simulink model "Cable_with_M_Inductance_Modelling_Study"  (R2024b)
settings: Solver=FixedStepDiscrete  StartTime=0.0  StopTime=5  FixedStep=1e-6  RelTol=1e-3
values from neighbouring files (symbols this model uses):
  Ccs1 = 733.62e-12    (= 7.3362e-10)    [Cable_Data_Inductance_Study.m]
  Ccs2 = 733.62e-12    (= 7.3362e-10)    [Cable_Data_Inductance_Study.m]
  Csg1 = 216.23e-12    (= 2.1623e-10)    [Cable_Data_Inductance_Study.m]
  Csg2 = 216.23e-12    (= 2.1623e-10)    [Cable_Data_Inductance_Study.m]
  Css = 93.23e-12    (= 9.323e-11)    [Cable_Data_Inductance_Study.m]
  L35 = 0.098e-6    (= 9.8e-08)    [Cable_Data_Inductance_Study.m]
  Lc1_total = Lc1 + Mcs1    (= 2.72e-07)    [Cable_Data_Inductance_Study.m]
  Lc2_total = Lc2 + Mcs2    (= 2.72e-07)    [Cable_Data_Inductance_Study.m]
  Len35_batt1_HVJB1_neg = 0.600    (= 0.6)    [Cable_Data_Inductance_Study.m]
  Len35_batt1_HVJB1_pos = 0.750    (= 0.75)    [Cable_Data_Inductance_Study.m]
  Len_parallel = min(Len35_batt1_HVJB1_pos,Len35_batt1_HVJB1_neg)    [Cable_Data_Inductance_Study.m]
  Ls1_eff = Ls1 + Mss_cal    [Cable_Data_Inductance_Study.m]
  Ls2_eff = Ls2 + Mss_cal    [Cable_Data_Inductance_Study.m]
  Mcs1 = 0.180e-6    (= 1.8e-07)    [Cable_Data_Inductance_Study.m]
  Mcs2 = 0.180e-6    (= 1.8e-07)    [Cable_Data_Inductance_Study.m]
  Rc1 = 0.38e-3    (= 0.00038)    [Cable_Data_Inductance_Study.m]
  Rc2 = 0.38e-3    (= 0.00038)    [Cable_Data_Inductance_Study.m]
  Rs1 = 2.55e-3    (= 0.00255)    [Cable_Data_Inductance_Study.m]
  Rs2 = 2.55e-3    (= 0.00255)    [Cable_Data_Inductance_Study.m]
undefined symbols (not defined in the file or in its folder): DiscIntNeverNeededParam, Lns95, Lps95
libraries: spsSeriesRLCBranchLib x18, spsCurrentMeasurementLib x7, spsMultimeterLib x6, spsVoltageMeasurementLib x5, eeGeneralControl x2, spsMutualInductanceLib x2, spsVariableResistorLib x1, spsGroundLib x1, spsDCVoltageSourceLib x1, spspowerguiLib x1
settings Model: PauseTimes=9  SnapshotBufferSize=100000000  SnapshotInterval=100  Creator=SUDHAK1  LastModifiedBy=SUDHAK1

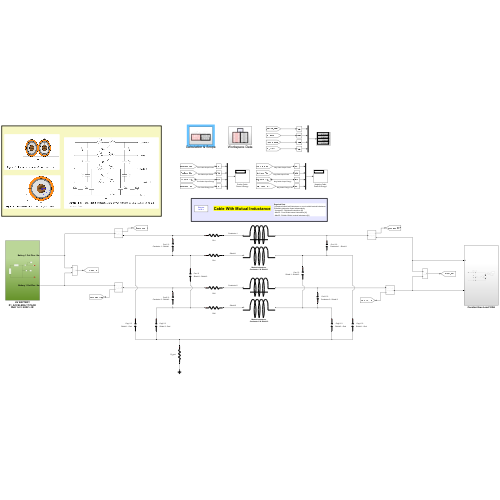
[thumbnail: Simulink's stored preview of the top-level diagram]
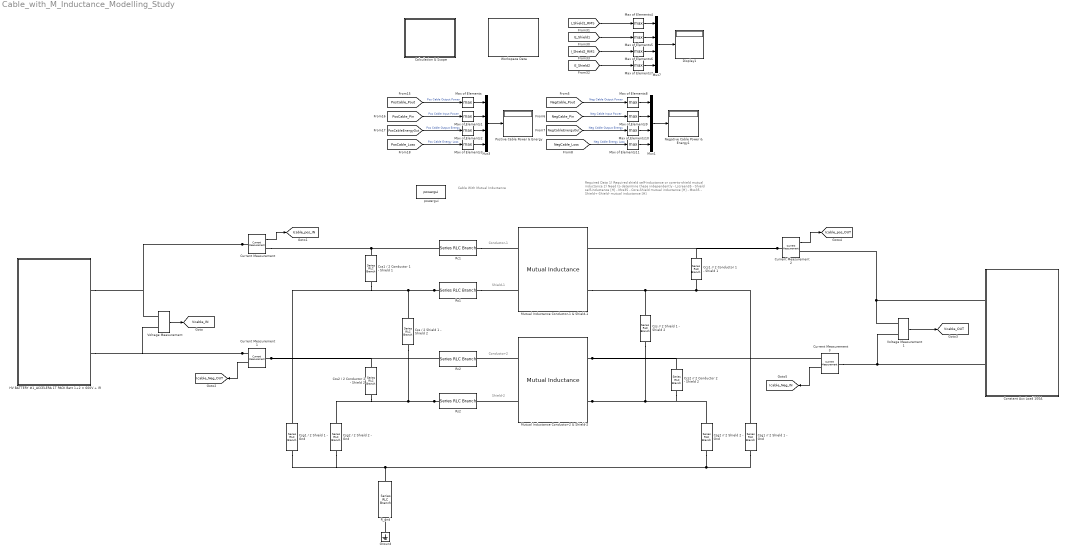
== system Cable_with_M_Inductance_Modelling_Study ==
  note: Cable With Mutual Inductance
  note: Shield-2
  note: Conductor-1
  note: Shield-1
  note: Required Data
      | 1) Required shield self-inductance or core-to-shield mutual inductance
      | 2) Need to determine these independently
      | - Lscreen35 - Shield self-inductance [H]
      | - Mcs35 - Core-Shield mutual inductance [H]
      | - Mss35 - Shield+-Shield- mutual inductance [H]
  note: Conductor-2
  " Ccs1 // 2 Conductor 1 - Shield 1" : spsSeriesRLCBranchLib/Series RLC Branch  LConnTagsString=__new0  RConnTagsString=__new0  BranchType=C  Resistance=1  Inductance=1e-3  SetiL0=off  InitialCurrent=0  Capacitance=(Ccs1/2)*Len35_batt1_HVJB1_pos  Setx0=off  InitialVoltage=0  Measurements=None
  " Ccs2 // 2 Conductor 2 - Shield 2" : spsSeriesRLCBranchLib/Series RLC Branch  LConnTagsString=__new0  RConnTagsString=__new0  BranchType=C  Resistance=1  Inductance=1e-3  SetiL0=off  InitialCurrent=0  Capacitance=(Ccs2/2)*Len35_batt1_HVJB1_neg  Setx0=off  InitialVoltage=0  Measurements=None
  " Csg1 // 2 Shield 1 - Gnd" : spsSeriesRLCBranchLib/Series RLC Branch  LConnTagsString=__new0  RConnTagsString=__new0  BranchType=C  Resistance=1  Inductance=1e-3  SetiL0=off  InitialCurrent=0  Capacitance=(Csg1/2)*Len35_batt1_HVJB1_pos  Setx0=off  InitialVoltage=0  Measurements=Branch voltage and current
  " Csg2 // 2 Shield 2 - Gnd" : spsSeriesRLCBranchLib/Series RLC Branch  LConnTagsString=__new0  RConnTagsString=__new0  BranchType=C  Resistance=1  Inductance=1e-3  SetiL0=off  InitialCurrent=0  Capacitance=(Csg2/2)*Len35_batt1_HVJB1_neg  Setx0=off  InitialVoltage=0  Measurements=Branch voltage and current
  " Css // 2 Shield 1 - Shield 2" : spsSeriesRLCBranchLib/Series RLC Branch  LConnTagsString=__new0  RConnTagsString=__new0  BranchType=C  Resistance=1  Inductance=1e-3  SetiL0=off  InitialCurrent=0  Capacitance=(Css/2)*Len_parallel  Setx0=off  InitialVoltage=0  Measurements=Branch voltage and current
  Calculation & Scope : Subsystem
  Ccs1 / 2 Conductor 1 - Shield 1 : spsSeriesRLCBranchLib/Series RLC Branch  LConnTagsString=__new0  RConnTagsString=__new0  BranchType=C  Resistance=1  Inductance=1e-3  SetiL0=off  InitialCurrent=0  Capacitance=(Ccs1/2)*Len35_batt1_HVJB1_pos  Setx0=off  InitialVoltage=0  Measurements=None
  Ccs2 / 2 Conductor 2 - Shield 2 : spsSeriesRLCBranchLib/Series RLC Branch  LConnTagsString=__new0  RConnTagsString=__new0  BranchType=C  Resistance=1  Inductance=1e-3  SetiL0=off  InitialCurrent=0  Capacitance=(Ccs2/2)*Len35_batt1_HVJB1_neg  Setx0=off  InitialVoltage=0  Measurements=None
  Constant Aux Load 100A : Subsystem
  Csg1 / 2 Shield 1 - Gnd : spsSeriesRLCBranchLib/Series RLC Branch  LConnTagsString=__new0  RConnTagsString=__new0  BranchType=C  Resistance=1  Inductance=1e-3  SetiL0=off  InitialCurrent=0  Capacitance=(Csg1/2)*Len35_batt1_HVJB1_pos  Setx0=off  InitialVoltage=0  Measurements=Branch voltage and current
  Csg2 / 2 Shield 2 - Gnd : spsSeriesRLCBranchLib/Series RLC Branch  LConnTagsString=__new0  RConnTagsString=__new0  BranchType=C  Resistance=1  Inductance=1e-3  SetiL0=off  InitialCurrent=0  Capacitance=(Csg2/2)*Len35_batt1_HVJB1_neg  Setx0=off  InitialVoltage=0  Measurements=Branch voltage and current
  Css / 2 Shield 1 - Shield 2 : spsSeriesRLCBranchLib/Series RLC Branch  LConnTagsString=__new0  RConnTagsString=__new0  BranchType=C  Resistance=1  Inductance=1e-3  SetiL0=off  InitialCurrent=0  Capacitance=(Css/2)*Len_parallel  Setx0=off  InitialVoltage=0  Measurements=Branch voltage and current
  Current Measurement{,1..3} (4 alike) : spsCurrentMeasurementLib/Current Measurement  PhasorSimulation=off  OutputType=Complex  PSBequivalent=0
  Display1 : Display
  Ground : spsGroundLib/Ground  LConnTagsString=a
  HV BATTERY #1_ACCELERA 1T PACK Batt 1+2 = 600V + IR : Subsystem
  Max of Elements{,1..11} (12 alike) : MinMax  Function=max
  Mutual Inductance Conductor-1 & Shield-1 : spsMutualInductanceLib/Mutual Inductance  LConnTagsString=a|b  RConnTagsString=A|B  TypeOfMutual=Two or three windings with equal mutual terms  NumberOfWindings=3  SelfImpedance1=[0 Lc1_total*Len35_batt1_HVJB1_pos]  SelfImpedance2=[0 Ls1_eff*Len35_batt1_HVJB1_pos]  ThreeWindings=off  SelfImpedance3=[ 1.1 1.1e-03]  MutualImpedance=[0 Mcs1*Len35_batt1_HVJB1_pos]  InductanceMatrix="[1.0 0.9  0.9 ;  0.9 1.0  0.9;  0.9 0.9 1.0 ] * 1e-3"  ResistanceMatrix="[1.0 0.9  0.9 ;  0.9 1.0  0.9;  0.9 0.9 1.0 ]"  Measurements=Winding voltages and currents
      settings: LibrarySourceBlock=sps_lib/Passives/Mutual Inductance
  Mutual Inductance Conductor-2 & Shield-2 : spsMutualInductanceLib/Mutual Inductance  LConnTagsString=a|b  RConnTagsString=A|B  TypeOfMutual=Two or three windings with equal mutual terms  NumberOfWindings=3  SelfImpedance1=[0 Lc2_total*Len35_batt1_HVJB1_neg]  SelfImpedance2=[0 Ls2_eff*Len35_batt1_HVJB1_neg]  ThreeWindings=off  SelfImpedance3=[ 1.1 1.1e-03]  MutualImpedance=[0 Mcs2*Len35_batt1_HVJB1_neg]  InductanceMatrix="[1.0 0.9  0.9 ;  0.9 1.0  0.9;  0.9 0.9 1.0 ] * 1e-3"  ResistanceMatrix="[1.0 0.9  0.9 ;  0.9 1.0  0.9;  0.9 0.9 1.0 ]"  Measurements=Winding voltages and currents
      settings: LibrarySourceBlock=sps_lib/Passives/Mutual Inductance
  Mux1 : Mux
  Mux3 : Mux
  Mux7 : Mux
  Negative Cable Power & Energy1 : Display
  Postive Cable Power & Energy : Display
  R_gnd : spsSeriesRLCBranchLib/Series RLC Branch  LConnTagsString=__new0  RConnTagsString=__new0  BranchType=R  Resistance=10e-03  Inductance=1e-3  SetiL0=off  InitialCurrent=0  Capacitance=1e-6  Setx0=off  InitialVoltage=0  Measurements=Branch voltage and current
  Rc1 : spsSeriesRLCBranchLib/Series RLC Branch  LConnTagsString=__new0  RConnTagsString=__new0  BranchType=R  Resistance=Rc1*Len35_batt1_HVJB1_pos  Inductance=L35*Len35_batt1_HVJB1_pos  SetiL0=off  InitialCurrent=0  Capacitance=1e-6  Setx0=off  InitialVoltage=0  Measurements=None
  Rc2 : spsSeriesRLCBranchLib/Series RLC Branch  LConnTagsString=__new0  RConnTagsString=__new0  BranchType=R  Resistance=Rc2*Len35_batt1_HVJB1_neg  Inductance=L35*Len35_batt1_HVJB1_pos  SetiL0=off  InitialCurrent=0  Capacitance=1e-6  Setx0=off  InitialVoltage=0  Measurements=None
  Rs1 : spsSeriesRLCBranchLib/Series RLC Branch  LConnTagsString=__new0  RConnTagsString=__new0  BranchType=R  Resistance=Rs1*Len35_batt1_HVJB1_pos  Inductance=Lps95*3.270  SetiL0=off  InitialCurrent=0  Capacitance=1e-6  Setx0=off  InitialVoltage=0  Measurements=None
  Rs2 : spsSeriesRLCBranchLib/Series RLC Branch  LConnTagsString=__new0  RConnTagsString=__new0  BranchType=R  Resistance=Rs2*Len35_batt1_HVJB1_neg  Inductance=Lns95*3.305  SetiL0=off  InitialCurrent=0  Capacitance=1e-6  Setx0=off  InitialVoltage=0  Measurements=None
  Voltage Measurement : spsVoltageMeasurementLib/Voltage Measurement  PhasorSimulation=off  OutputType=Complex  PSBequivalent=0
  Voltage Measurement1 : spsVoltageMeasurementLib/Voltage Measurement  PhasorSimulation=off  OutputType=Complex  PSBequivalent=0
  Workspace Data : Subsystem
  powergui : spspowerguiLib/powergui  Priority=1  SimulationMode=Discrete  SampleTime=1e-6  frequency=60  Iterations=50  frequencyindice=0  Pbase=100e6  ErrMax=1e-4  UnitsV=kV  UnitsW=MW  buscounter=0  FunctionMessages=off  echomessages=off  EnableUseOfTLC=off  CurrentSourceSwitches=off  DisableSnubberDevices=off  DisableRonSwitches=off  DisableVfSwitches=off  DisplayEquations=off  AutomaticDiscreteSolvers=off  SolverType=Tustin/Backward Euler (TBE)  Interpol=off  ExternalGateDelay=off  methode=off  Ts=100  x0status=blocks  SPID=on  SwTol=0  HookPort=off  NonlinearTolerance=1e-4  nMaxIteration=100  ContinueOnMaxIteration=off  RestoreLinks=warning  ResistiveCurrentMeasurement=off  Frange=[0:2:500]  Ylog=off  Xlog=on  ShowGrid=off  save=off  variable=ZData  structure=0  ZoomFFT=off  StartTime=0.0  cycles=1  DisplayStyle=1  fundamental=60  FreqAxis=off  MaxFrequency=1000  frequencyindicesteady=1  RmsSteady=1  display=off
  tag scope: Icable_Neg_IN=global, Icable_Neg_OUT=global, Icable_pos_IN=global, Icable_pos_OUT=global, Vcable_IN=global, Vcable_OUT=global
  wires:
  Current Measurement2/1 -> [Icable_pos_OUT]
  Current Measurement3/1 -> [Icable_Neg_IN]
  Voltage Measurement1/1 -> [Vcable_OUT]
  Current Measurement1/1 -> [Icable_Neg_OUT]
  Voltage Measurement/1 -> [Vcable_IN]
  Current Measurement/1 -> [Icable_pos_IN]
  Max of Elements4/1 -> Mux7/1
  Max of Elements5/1 -> Mux7/2
  Mux7/1 -> Display1/1
  [I_Shield1_RMS] -> Max of Elements4/1
  [E_Shield1] -> Max of Elements5/1
  Max of Elements6/1 -> Mux7/3
  Max of Elements7/1 -> Mux7/4
  [I_Shield2_RMS] -> Max of Elements6/1
  [E_Shield2] -> Max of Elements7/1
  [NegCable_Loss] -> Max of Elements11/1  "Neg Cable Energy Loss"
  [NegCableEnergyOut] -> Max of Elements10/1  "Neg Cable Output Energy"
  [PosCable_Loss] -> Max of Elements3/1  "Pos Cable Energy Loss"
  [PosCableEnergyOut] -> Max of Elements2/1  "Pos Cable Output Energy"
  [PosCable_Pout] -> Max of Elements/1  "Pos Cable Output Power"
  [NegCable_Pout] -> Max of Elements8/1  "Neg Cable Output Power"
  [NegCable_Pin] -> Max of Elements9/1  "Neg Cable Input Power"
  [PosCable_Pin] -> Max of Elements1/1  "Pos Cable Input Power"
  Max of Elements3/1 -> Mux3/4
  Max of Elements/1 -> Mux3/1
  Mux3/1 -> Postive Cable Power & Energy/1
  Max of Elements1/1 -> Mux3/2
  Max of Elements2/1 -> Mux3/3
  Max of Elements10/1 -> Mux1/3
  Max of Elements9/1 -> Mux1/2
  Max of Elements8/1 -> Mux1/1
  Mux1/1 -> Negative Cable Power & Energy1/1
  Max of Elements11/1 -> Mux1/4
  connections:
  Mutual Inductance Conductor-2 & Shield-2/RConn1 -- Current Measurement3/RConn1 -- " Ccs2 // 2 Conductor 2 - Shield 2"/RConn1
  Current Measurement1/RConn1 -- HV BATTERY #1_ACCELERA 1T PACK Batt 1+2 = 600V + IR/RConn2 -- Voltage Measurement/LConn2
  Current Measurement1/LConn1 -- Rc2/LConn1 -- Ccs2 / 2 Conductor 2 - Shield 2/LConn1
  Voltage Measurement1/LConn1 -- Constant Aux Load 100A/RConn1 -- Current Measurement2/RConn1
  Rs1/LConn1 -- Ccs1 / 2 Conductor 1 - Shield 1/RConn1 -- Csg1 / 2 Shield 1 - Gnd/LConn1 -- Css / 2 Shield 1 - Shield 2/LConn1
  Current Measurement/LConn1 -- Voltage Measurement/LConn1 -- HV BATTERY #1_ACCELERA 1T PACK Batt 1+2 = 600V + IR/RConn1
  Rs2/LConn1 -- Csg2 / 2 Shield 2 - Gnd/LConn1 -- Ccs2 / 2 Conductor 2 - Shield 2/RConn1 -- Css / 2 Shield 1 - Shield 2/RConn1
  Mutual Inductance Conductor-2 & Shield-2/RConn2 -- " Csg2 // 2 Shield 2 - Gnd"/LConn1 -- " Ccs2 // 2 Conductor 2 - Shield 2"/LConn1 -- " Css // 2 Shield 1 - Shield 2"/RConn1
  R_gnd/LConn1 -- Csg2 / 2 Shield 2 - Gnd/RConn1 -- Csg1 / 2 Shield 1 - Gnd/RConn1 -- " Csg2 // 2 Shield 2 - Gnd"/RConn1 -- " Csg1 // 2 Shield 1 - Gnd"/RConn1
  Current Measurement/RConn1 -- Rc1/LConn1 -- Ccs1 / 2 Conductor 1 - Shield 1/LConn1
  " Css // 2 Shield 1 - Shield 2"/LConn1 -- Mutual Inductance Conductor-1 & Shield-1/RConn2 -- " Csg1 // 2 Shield 1 - Gnd"/LConn1 -- " Ccs1 // 2 Conductor 1 - Shield 1"/RConn1
  Current Measurement3/LConn1 -- Constant Aux Load 100A/RConn2 -- Voltage Measurement1/LConn2
  Current Measurement2/LConn1 -- Mutual Inductance Conductor-1 & Shield-1/RConn1 -- " Ccs1 // 2 Conductor 1 - Shield 1"/LConn1
  Rs1/RConn1 -- Mutual Inductance Conductor-1 & Shield-1/LConn2
  Mutual Inductance Conductor-2 & Shield-2/LConn1 -- Rc2/RConn1
  Rc1/RConn1 -- Mutual Inductance Conductor-1 & Shield-1/LConn1
  Ground/LConn1 -- R_gnd/RConn1
  Mutual Inductance Conductor-2 & Shield-2/LConn2 -- Rs2/RConn1

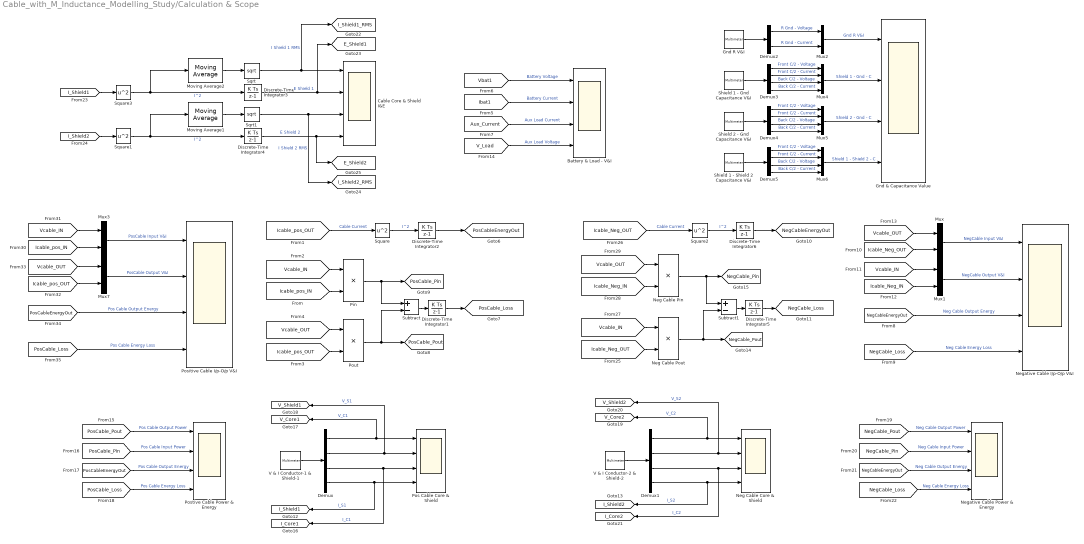
== system Cable_with_M_Inductance_Modelling_Study/Calculation & Scope ==
  Battery & Load - V&I : Scope  NumInputPorts=4
  Cable Core & Shield  I&E : Scope  NumInputPorts=4
  Demux{,1,3..5} (5 alike) : Demux
  Demux2 : Demux  Outputs=2
  Discrete-Time Integrator{1..6} (6 alike) : DiscreteIntegrator  SampleTime=-1  ICPrevOutput=DiscIntNeverNeededParam  ICPrevScaledInput=DiscIntNeverNeededParam
  Gnd & Capacitance Value : Scope  NumInputPorts=4
  Gnd R V&I : spsMultimeterLib/Multimeter  L=22  sel=[7 18]  yselected={}  Gain=[1 1]  OutputType=Complex  PlotAtSimulationStop=off  PhasorSimulation=off
  Moving Average1 : eeGeneralControl/Moving Average  VariantControl=Variant1  LabelModeActiveChoice=Discrete  f=60  x0=0  BufferSize=8192  Ts=-1
      settings: LibrarySourceBlock=ee_sl_lib/General Control/Moving Average
  Moving Average2 : eeGeneralControl/Moving Average  VariantControl=Variant1  LabelModeActiveChoice=Discrete  f=60  x0=0  BufferSize=8192  Ts=-1
      settings: LibrarySourceBlock=ee_sl_lib/General Control/Moving Average
  Mux{,1..3,7} (5 alike) : Mux  Inputs=2
  Mux4 : Mux
  Mux5 : Mux
  Mux6 : Mux
  Neg Cable Core & Shield : Scope  NumInputPorts=4
  Neg Cable Pin : Product
  Neg Cable Pout : Product
  Negative Cable Power & Energy : Scope  NumInputPorts=4
  Negative Cable I/p-O/p V&I : Scope  NumInputPorts=4
  Pin : Product
  Pos Cable Core & Shield : Scope  NumInputPorts=4
  Positive Cable I/p-O/p V&I : Scope  NumInputPorts=4
  Postive Cable Power & Energy : Scope  NumInputPorts=4
  Pout : Product
  Shield 1 - Gnd Capacitance V&I : spsMultimeterLib/Multimeter  L=22  sel=[4 15 1 12]  yselected={}  Gain=[1 1 1 1]  OutputType=Complex  PlotAtSimulationStop=off  PhasorSimulation=off
  Shield 1 - Shield 2 Capacitance V&I : spsMultimeterLib/Multimeter  L=22  sel=[6 17 3 14]  yselected={}  Gain=[1 1 1 1]  OutputType=Complex  PlotAtSimulationStop=off  PhasorSimulation=off
  Shield 2 - Gnd Capacitance V&I : spsMultimeterLib/Multimeter  L=22  sel=[5 16 2 13]  yselected={}  Gain=[1 1 1 1]  OutputType=Complex  PlotAtSimulationStop=off  PhasorSimulation=off
  Sqrt : Sqrt
  Sqrt1 : Sqrt
  Square{,1..3} (4 alike) : Math  Operator=square
  Subtract : Sum  Inputs=+-
  Subtract1 : Sum  Inputs=+-
  V & I Conductor-1 & Shield-1 : spsMultimeterLib/Multimeter  L=22  sel=[8 9 19 20]  yselected={}  Gain=[1 1 1 1]  OutputType=Complex  PlotAtSimulationStop=off  PhasorSimulation=off
  V & I Conductor-2 & Shield-2 : spsMultimeterLib/Multimeter  L=22  sel=[10 11 21 22]  yselected={}  Gain=[1 1 1 1]  OutputType=Complex  PlotAtSimulationStop=off  PhasorSimulation=off
  tag scope: E_Shield1=global, E_Shield2=global, I_Core1=global, I_Core2=global, I_Shield1=global, I_Shield1_RMS=global, I_Shield2=global, I_Shield2_RMS=global, NegCableEnergyOut=global, NegCable_Loss=global, NegCable_Pin=global, NegCable_Pout=global, PosCableEnergyOut=global, PosCable_Loss=global, PosCable_Pin=global, PosCable_Pout=global, V_Core1=global, V_Core2=global, V_Shield1=global, V_Shield2=global
  wires:
  [NegCableEnergyOut] -> Negative Cable I/p-O/p V&I/3  "Neg Cable Output Energy"
  Moving Average2/1 -> Sqrt/1
  Mux6/1 -> Gnd & Capacitance Value/4  "Shield 1 - Shield 2 - C"
  Square/1 -> Discrete-Time Integrator2/1  "I^2"
  Demux4/2 -> Mux5/2  "Front C/2 - Current"
  Mux4/1 -> Gnd & Capacitance Value/2  "Shield 1 - Gnd - C"
  [Icable_pos_IN] -> Pin/2
  Demux/4 -> [I_Shield1], Pos Cable Core & Shield/4  "I_S1"
  [PosCableEnergyOut] -> Postive Cable Power & Energy/3  "Pos Cable Output Energy"
  Demux5/2 -> Mux6/2  "Front C/2 - Current"
  Shield 1 - Shield 2 Capacitance V&I/1 -> Demux5/1
  Mux5/1 -> Gnd & Capacitance Value/3  "Shield 2 - Gnd - C"
  Shield 2 - Gnd Capacitance V&I/1 -> Demux4/1
  [Icable_pos_OUT] -> Pout/2
  Demux3/2 -> Mux4/2  "Front C/2 - Current"
  Demux1/2 -> Neg Cable Core & Shield/2, [V_Shield2]  "V_S2"
  [Icable_pos_OUT] -> Square/1  "Cable Current"
  Moving Average1/1 -> Sqrt1/1
  Discrete-Time Integrator3/1 -> [E_Shield1], Cable Core & Shield  I&E/2  "E Shield 1"
  Demux1/1 -> [V_Core2], Neg Cable Core & Shield/1  "V_C2"
  Demux/1 -> Pos Cable Core & Shield/1, [V_Core1]  "V_C1"
  Pin/1 -> [PosCable_Pin], Subtract/1
  Demux4/4 -> Mux5/4  "Back C/2 - Current"
  [Vcable_OUT] -> Pout/1
  Mux/1 -> Negative Cable I/p-O/p V&I/1  "NegCable Input V&I"
  V & I Conductor-1 & Shield-1/1 -> Demux/1
  [Aux_Current] -> Battery & Load - V&I/3  "Aux Load Current"
  [V_Load] -> Battery & Load - V&I/4  "Aux Load Voltage"
  [Icable_Neg_OUT] -> Mux/2
  Demux4/1 -> Mux5/1  "Front C/2 - Voltage"
  Discrete-Time Integrator4/1 -> Cable Core & Shield  I&E/4, [E_Shield2]  "E Shield 2"
  Square3/1 -> Discrete-Time Integrator3/1, Moving Average2/1  "I^2"
  [I_Shield1] -> Square3/1
  [Vbat1] -> Battery & Load - V&I/1  "Battery Voltage"
  Discrete-Time Integrator1/1 -> [PosCable_Loss]
  Sqrt1/1 -> Cable Core & Shield  I&E/3, [I_Shield2_RMS]  "I Shield 2 RMS"
  Demux5/4 -> Mux6/4  "Back C/2 - Current"
  Demux4/3 -> Mux5/3  "Back C/2 - Voltage"
  [Vcable_IN] -> Neg Cable Pout/1
  Demux2/2 -> Mux2/2  "R Gnd - Current"
  [NegCable_Loss] -> Negative Cable I/p-O/p V&I/4  "Neg Cable Energy Loss"
  Subtract/1 -> Discrete-Time Integrator1/1
  Demux5/1 -> Mux6/1  "Front C/2 - Voltage"
  Shield 1 - Gnd Capacitance V&I/1 -> Demux3/1
  Pout/1 -> Subtract/2, [PosCable_Pout]
  [Icable_Neg_OUT] -> Square2/1  "Cable Current"
  [PosCable_Pin] -> Postive Cable Power & Energy/2  "Pos Cable Input Power"
  Demux/2 -> Pos Cable Core & Shield/2, [V_Shield1]  "V_S1"
  Demux5/3 -> Mux6/3  "Back C/2 - Voltage"
  Demux2/1 -> Mux2/1  "R Gnd - Voltage"
  Mux2/1 -> Gnd & Capacitance Value/1  "Gnd R V&I"
  [I_Shield2] -> Square1/1
  Demux/3 -> [I_Core1], Pos Cable Core & Shield/3  "I_C1"
  Mux1/1 -> Negative Cable I/p-O/p V&I/2  "NegCable Output V&I"
  Demux3/3 -> Mux4/3  "Back C/2 - Voltage"
  Discrete-Time Integrator2/1 -> [PosCableEnergyOut]
  [Vcable_IN] -> Pin/1
  Gnd R V&I/1 -> Demux2/1
  Demux3/1 -> Mux4/1  "Front C/2 - Voltage"
  Square1/1 -> Discrete-Time Integrator4/1, Moving Average1/1  "I^2"
  [Icable_Neg_IN] -> Mux1/2
  [PosCable_Pout] -> Postive Cable Power & Energy/1  "Pos Cable Output Power"
  [PosCable_Loss] -> Postive Cable Power & Energy/4  "Pos Cable Energy Loss"
  Demux1/3 -> [I_Core2], Neg Cable Core & Shield/3  "I_C2"
  Demux1/4 -> [I_Shield2], Neg Cable Core & Shield/4  "I_S2"
  V & I Conductor-2 & Shield-2/1 -> Demux1/1
  [Ibat1] -> Battery & Load - V&I/2  "Battery Current"
  Sqrt/1 -> Cable Core & Shield  I&E/1, [I_Shield1_RMS]  "I Shield 1 RMS"
  Demux3/4 -> Mux4/4  "Back C/2 - Current"
  Subtract1/1 -> Discrete-Time Integrator5/1
  Discrete-Time Integrator5/1 -> [NegCable_Loss]
  Neg Cable Pout/1 -> Subtract1/2, [NegCable_Pout]
  Discrete-Time Integrator6/1 -> [NegCableEnergyOut]
  [Vcable_OUT] -> Neg Cable Pin/1
  Neg Cable Pin/1 -> Subtract1/1, [NegCable_Pin]
  [Icable_Neg_IN] -> Neg Cable Pin/2
  [Icable_Neg_OUT] -> Neg Cable Pout/2
  Square2/1 -> Discrete-Time Integrator6/1  "I^2"
  [NegCable_Loss] -> Negative Cable Power & Energy/4  "Neg Cable Energy Loss"
  [NegCableEnergyOut] -> Negative Cable Power & Energy/3  "Neg Cable Output Energy"
  [NegCable_Pout] -> Negative Cable Power & Energy/1  "Neg Cable Output Power"
  [NegCable_Pin] -> Negative Cable Power & Energy/2  "Neg Cable Input Power"
  [Icable_pos_IN] -> Mux3/2
  [Vcable_IN] -> Mux3/1
  [Icable_pos_OUT] -> Mux7/2
  [PosCable_Loss] -> Positive Cable I/p-O/p V&I/4  "Pos Cable Energy Loss"
  Mux3/1 -> Positive Cable I/p-O/p V&I/1  "PosCable Input V&I"
  Mux7/1 -> Positive Cable I/p-O/p V&I/2  "PosCable Output V&I"
  [Vcable_OUT] -> Mux7/1
  [PosCableEnergyOut] -> Positive Cable I/p-O/p V&I/3  "Pos Cable Output Energy"
  [Vcable_IN] -> Mux1/1
  [Vcable_OUT] -> Mux/1

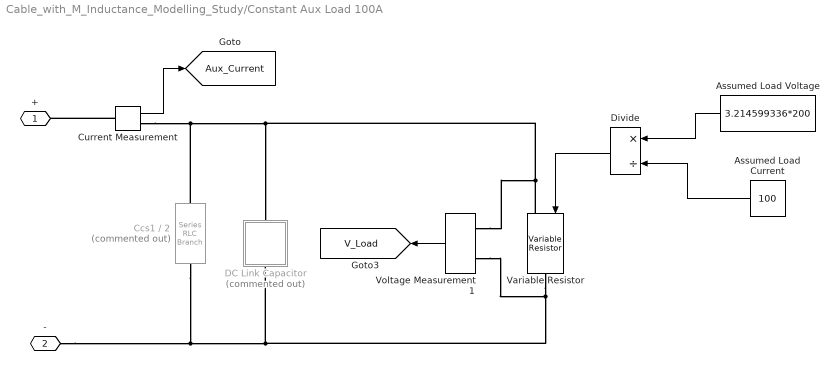
== system Cable_with_M_Inductance_Modelling_Study/Constant Aux Load 100A ==
  " Ccs1 / 2" : spsSeriesRLCBranchLib/Series RLC Branch  Commented=on  LConnTagsString=__new0  RConnTagsString=__new0  BranchType=R  Resistance=1  Inductance=1e-3  SetiL0=off  InitialCurrent=0  Capacitance=Ccs1/2  Setx0=off  InitialVoltage=0  Measurements=None
  Assumed Load Current : Constant  Value=100
  Assumed Load Voltage : Constant  Value=3.214599336*200
  Current Measurement : spsCurrentMeasurementLib/Current Measurement  PhasorSimulation=off  OutputType=Complex  PSBequivalent=0
  DC Link Capacitor : Subsystem  Commented=on
      settings: PortSchema="{\"entries\":[{\"content\":{\"sides\":[{\"content\":{},\"type\":\"ConnectorPlacement.EquallySpacedRectSide\",\"uuid\":\"a9c9044e-480e-49f2-9d9a-ad6fbdeb65df\"},{\"content\":{\"side\":\"RIGHT\"},\"type\":\"ConnectorPlacement.EquallySpacedRectSide\",\"uuid\":\"db4a4fc7-6a64-44bf-88d6-5d8062a8668f\"},{\"content\":{\"connectorIds\":[\"LConn1\"],\"side\":\"TOP\"},\"type\":\"ConnectorPlacement.EquallySpacedRectSide\",\"uuid\":\"c4fbeb8e-5c35-4874-aa8f-a5810cded374\"},{\"content\":{\"connectorIds\":[\"RConn1\"],\"side\":\"BOTTOM\"},\"type\":\"ConnectorPlacement.EquallySpacedRectSide\",\"uuid\":\"95f71b14-027a-489a-83bf-19494ef52344\"}]},\"type\":\"ConnectorPlacement.EquallySpacedConnector\",\"uuid\":\"3c0edebe-2bcc-4259-9d3a-139f17972178\"}],\"packageUris\":[\"http://schema.mathworks.com/mf0/Connector/R2020b\"],\"version\":\"1.0\"}"
  Divide : Product  Inputs=*/
  Variable Resistor : spsVariableResistorLib/Variable Resistor  Rabsmin=1e-3
  Voltage Measurement1 : spsVoltageMeasurementLib/Voltage Measurement  PhasorSimulation=off  OutputType=Complex  PSBequivalent=0
  + : PMIOPort  Side=Right
  - : PMIOPort  Port=2  Side=Right
  tag scope: Aux_Current=global, V_Load=global
  wires:
  Current Measurement/1 -> [Aux_Current]
  Divide/1 -> Variable Resistor/1
  Assumed Load Current/1 -> Divide/2
  Assumed Load Voltage/1 -> Divide/1
  Voltage Measurement1/1 -> [V_Load]
  connections:
  Current Measurement/LConn1 -- +/RConn1
  Current Measurement/RConn1 -- " Ccs1 / 2"/LConn1 -- Variable Resistor/LConn1 -- Voltage Measurement1/LConn1 -- DC Link Capacitor/RConn1
  -/RConn1 -- Voltage Measurement1/LConn2 -- Variable Resistor/RConn1 -- DC Link Capacitor/LConn1 -- " Ccs1 / 2"/RConn1

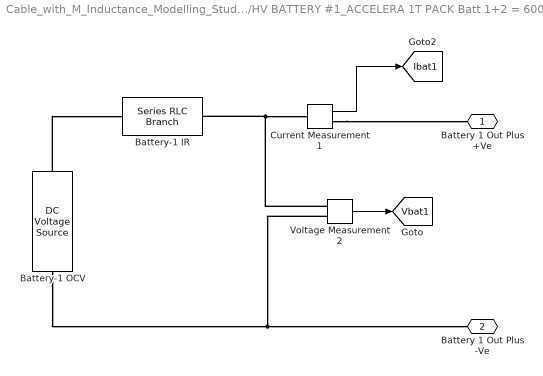
== system Cable_with_M_Inductance_Modelling_Study/HV BATTERY #1_ACCELERA 1T PACK Batt 1+2 = 600V + IR ==
  Battery-1 IR : spsSeriesRLCBranchLib/Series RLC Branch  LConnTagsString=__new0  RConnTagsString=__new0  BranchType=R  Resistance=(2.14417*200)*1e-3  Inductance=1e-3  SetiL0=off  InitialCurrent=0  Capacitance=1e-6  Setx0=off  InitialVoltage=0  Measurements=None
  Battery-1 OCV : spsDCVoltageSourceLib/DC Voltage Source  Amplitude=3.214599336*200  Measurements=None
  Current Measurement1 : spsCurrentMeasurementLib/Current Measurement  PhasorSimulation=off  OutputType=Complex  PSBequivalent=0
  Voltage Measurement2 : spsVoltageMeasurementLib/Voltage Measurement  PhasorSimulation=off  OutputType=Complex  PSBequivalent=0
  Battery 1 Out Plus +Ve : PMIOPort  Side=Right
  Battery 1 Out Plus -Ve : PMIOPort  Port=2  Side=Right
  tag scope: Ibat1=global, Vbat1=global
  wires:
  Voltage Measurement2/1 -> [Vbat1]
  Current Measurement1/1 -> [Ibat1]
  connections:
  Voltage Measurement2/LConn2 -- Battery-1 OCV/LConn1 -- Battery 1 Out Plus -Ve/RConn1
  Voltage Measurement2/LConn1 -- Current Measurement1/LConn1 -- Battery-1 IR/RConn1
  Current Measurement1/RConn1 -- Battery 1 Out Plus +Ve/RConn1
  Battery-1 OCV/RConn1 -- Battery-1 IR/LConn1

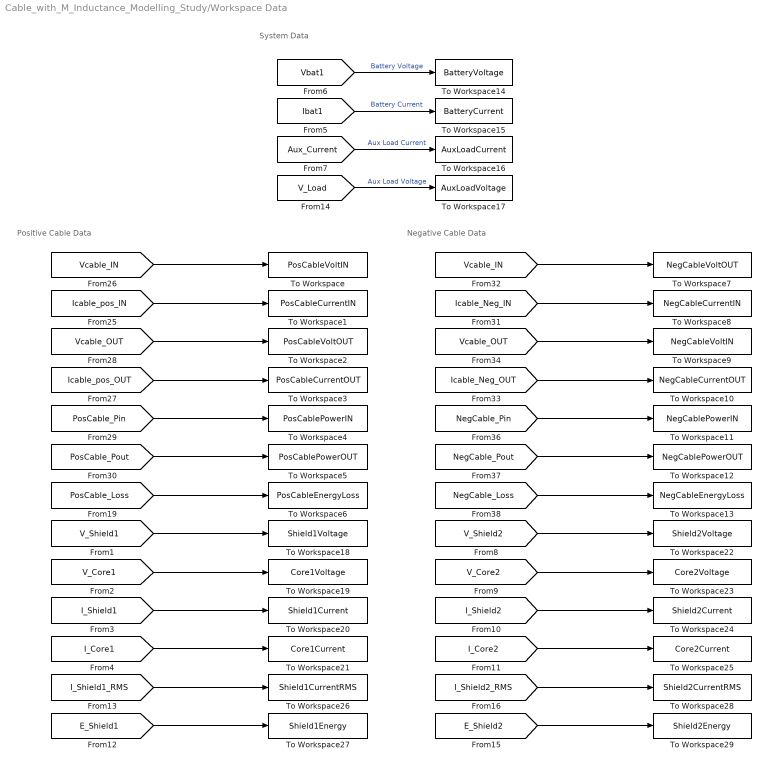
== system Cable_with_M_Inductance_Modelling_Study/Workspace Data ==
  note: System Data
  note: Negative Cable Data
  note: Positive Cable Data
  To Workspace : ToWorkspace  VariableName=PosCableVoltIN  SaveFormat=Timeseries  SampleTime=-1
  To Workspace1 : ToWorkspace  VariableName=PosCableCurrentIN  SaveFormat=Timeseries  SampleTime=-1
  To Workspace10 : ToWorkspace  VariableName=NegCableCurrentOUT  SaveFormat=Timeseries  SampleTime=-1
  To Workspace11 : ToWorkspace  VariableName=NegCablePowerIN  SaveFormat=Timeseries  SampleTime=-1
  To Workspace12 : ToWorkspace  VariableName=NegCablePowerOUT  SaveFormat=Timeseries  SampleTime=-1
  To Workspace13 : ToWorkspace  VariableName=NegCableEnergyLoss  SaveFormat=Timeseries  SampleTime=-1
  To Workspace14 : ToWorkspace  VariableName=BatteryVoltage  SaveFormat=Timeseries  SampleTime=-1
  To Workspace15 : ToWorkspace  VariableName=BatteryCurrent  SaveFormat=Timeseries  SampleTime=-1
  To Workspace16 : ToWorkspace  VariableName=AuxLoadCurrent  SaveFormat=Timeseries  SampleTime=-1
  To Workspace17 : ToWorkspace  VariableName=AuxLoadVoltage  SaveFormat=Timeseries  SampleTime=-1
  To Workspace18 : ToWorkspace  VariableName=Shield1Voltage  SaveFormat=Timeseries  SampleTime=-1
  To Workspace19 : ToWorkspace  VariableName=Core1Voltage  SaveFormat=Timeseries  SampleTime=-1
  To Workspace2 : ToWorkspace  VariableName=PosCableVoltOUT  SaveFormat=Timeseries  SampleTime=-1
  To Workspace20 : ToWorkspace  VariableName=Shield1Current  SaveFormat=Timeseries  SampleTime=-1
  To Workspace21 : ToWorkspace  VariableName=Core1Current  SaveFormat=Timeseries  SampleTime=-1
  To Workspace22 : ToWorkspace  VariableName=Shield2Voltage  SaveFormat=Timeseries  SampleTime=-1
  To Workspace23 : ToWorkspace  VariableName=Core2Voltage  SaveFormat=Timeseries  SampleTime=-1
  To Workspace24 : ToWorkspace  VariableName=Shield2Current  SaveFormat=Timeseries  SampleTime=-1
  To Workspace25 : ToWorkspace  VariableName=Core2Current  SaveFormat=Timeseries  SampleTime=-1
  To Workspace26 : ToWorkspace  VariableName=Shield1CurrentRMS  SaveFormat=Timeseries  SampleTime=-1
  To Workspace27 : ToWorkspace  VariableName=Shield1Energy  SaveFormat=Timeseries  SampleTime=-1
  To Workspace28 : ToWorkspace  VariableName=Shield2CurrentRMS  SaveFormat=Timeseries  SampleTime=-1
  To Workspace29 : ToWorkspace  VariableName=Shield2Energy  SaveFormat=Timeseries  SampleTime=-1
  To Workspace3 : ToWorkspace  VariableName=PosCableCurrentOUT  SaveFormat=Timeseries  SampleTime=-1
  To Workspace4 : ToWorkspace  VariableName=PosCablePowerIN  SaveFormat=Timeseries  SampleTime=-1
  To Workspace5 : ToWorkspace  VariableName=PosCablePowerOUT  SaveFormat=Timeseries  SampleTime=-1
  To Workspace6 : ToWorkspace  VariableName=PosCableEnergyLoss  SaveFormat=Timeseries  SampleTime=-1
  To Workspace7 : ToWorkspace  VariableName=NegCableVoltOUT  SaveFormat=Timeseries  SampleTime=-1
  To Workspace8 : ToWorkspace  VariableName=NegCableCurrentIN  SaveFormat=Timeseries  SampleTime=-1
  To Workspace9 : ToWorkspace  VariableName=NegCableVoltIN  SaveFormat=Timeseries  SampleTime=-1
  wires:
  [Ibat1] -> To Workspace15/1  "Battery Current"
  [Vbat1] -> To Workspace14/1  "Battery Voltage"
  [V_Load] -> To Workspace17/1  "Aux Load Voltage"
  [Aux_Current] -> To Workspace16/1  "Aux Load Current"
  [Vcable_IN] -> To Workspace/1
  [Icable_pos_IN] -> To Workspace1/1
  [Vcable_OUT] -> To Workspace2/1
  [Icable_pos_OUT] -> To Workspace3/1
  [PosCable_Pin] -> To Workspace4/1
  [PosCable_Pout] -> To Workspace5/1
  [PosCable_Loss] -> To Workspace6/1
  [NegCable_Loss] -> To Workspace13/1
  [NegCable_Pin] -> To Workspace11/1
  [Vcable_IN] -> To Workspace7/1
  [Vcable_OUT] -> To Workspace9/1
  [Icable_Neg_IN] -> To Workspace8/1
  [NegCable_Pout] -> To Workspace12/1
  [Icable_Neg_OUT] -> To Workspace10/1
  [V_Shield1] -> To Workspace18/1
  [V_Core1] -> To Workspace19/1
  [I_Shield1] -> To Workspace20/1
  [I_Core1] -> To Workspace21/1
  [V_Shield2] -> To Workspace22/1
  [V_Core2] -> To Workspace23/1
  [I_Shield2] -> To Workspace24/1
  [I_Core2] -> To Workspace25/1
  [I_Shield2_RMS] -> To Workspace28/1
  [E_Shield1] -> To Workspace27/1
  [I_Shield1_RMS] -> To Workspace26/1
  [E_Shield2] -> To Workspace29/1

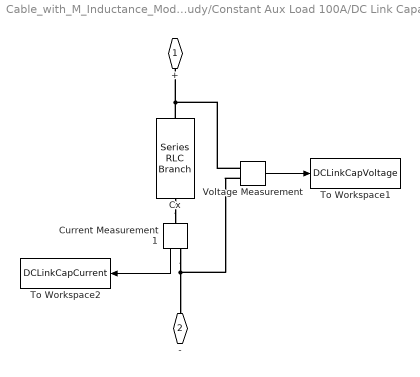
== system Cable_with_M_Inductance_Modelling_Study/Constant Aux Load 100A/DC Link Capacitor ==
  Current Measurement1 : spsCurrentMeasurementLib/Current Measurement  PhasorSimulation=off  OutputType=Complex  PSBequivalent=0
  Cx : spsSeriesRLCBranchLib/Series RLC Branch  LConnTagsString=__new0  RConnTagsString=__new0  BranchType=C  Resistance=0.5  Inductance=1e-3  SetiL0=off  InitialCurrent=0  Capacitance=2e-3  Setx0=on  InitialVoltage=Cx_Vs  Measurements=Branch voltage and current
  To Workspace1 : ToWorkspace  VariableName=DCLinkCapVoltage  SaveFormat=Timeseries  SampleTime=-1
  To Workspace2 : ToWorkspace  VariableName=DCLinkCapCurrent  SaveFormat=Timeseries  SampleTime=-1
  Voltage Measurement : spsVoltageMeasurementLib/Voltage Measurement  PhasorSimulation=off  OutputType=Complex  PSBequivalent=0
  + : PMIOPort  Side=Left
  - : PMIOPort  Port=2  Side=Right
  wires:
  Voltage Measurement/1 -> To Workspace1/1
  Current Measurement1/1 -> To Workspace2/1
  connections:
  Current Measurement1/RConn1 -- -/RConn1 -- Voltage Measurement/LConn2
  Cx/RConn1 -- Current Measurement1/LConn1
  Voltage Measurement/LConn1 -- +/RConn1 -- Cx/LConn1
